simulink model "Hopper_GMEKF"  (R2026a)
settings: Solver=FixedStepAuto
settings Model: DataDictionary=NavigationDictionary.sldd  Creator=David  LastModifiedBy=David

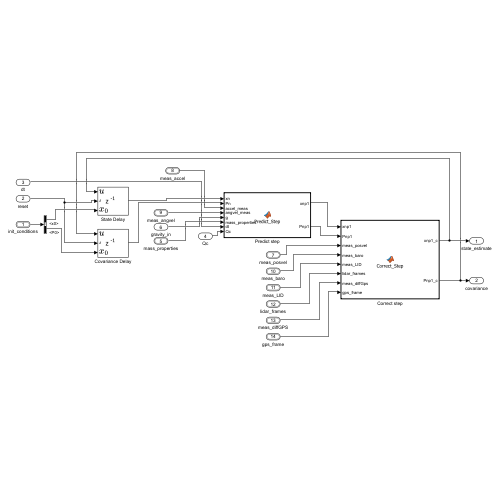
[thumbnail: Simulink's stored preview of the top-level diagram]
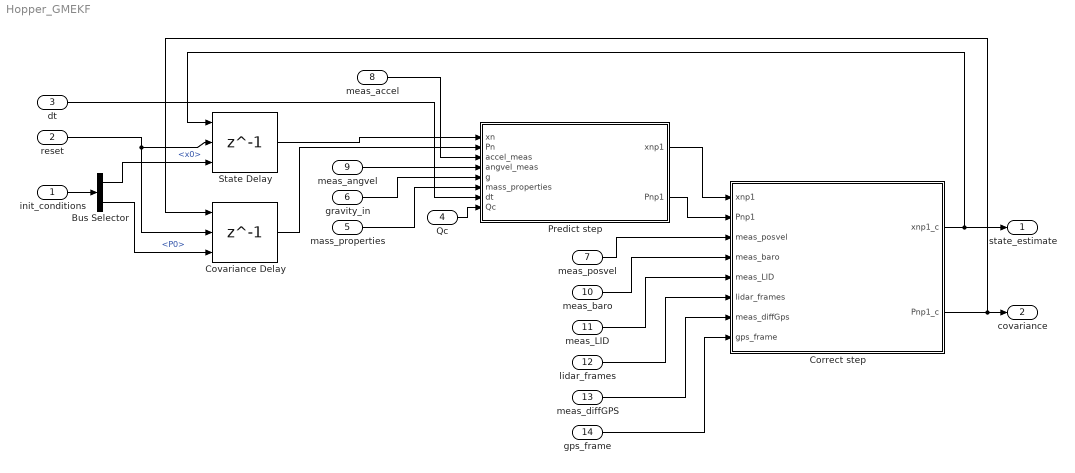
== system Hopper_GMEKF ==
  init_conditions : Inport  OutDataTypeStr=Bus: InitConditions
  reset : Inport  Port=2  OutDataTypeStr=ValueType: reset
  dt : Inport  Port=3  OutDataTypeStr=ValueType: timestep
  Qc : Inport  Port=4  OutDataTypeStr=ValueType: Qc
  mass_properties : Inport  Port=5  OutDataTypeStr=Bus: massProperties
  gravity_in : Inport  Port=6  OutDataTypeStr=ValueType: gravity
  meas_posvel : Inport  Port=7  OutDataTypeStr=Bus: gpsBus
  meas_accel : Inport  Port=8  OutDataTypeStr=Bus: accelBus
  meas_angvel : Inport  Port=9  OutDataTypeStr=Bus: angvelBus
  meas_baro : Inport  Port=10  OutDataTypeStr=Bus: baroBus
  meas_LID : Inport  Port=11  OutDataTypeStr=Bus: lidarBus
  lidar_frames : Inport  Port=12  OutDataTypeStr=Bus: lidarFrameBus
  meas_diffGPS : Inport  Port=13  OutDataTypeStr=Bus: diffGpsBus
  gps_frame : Inport  Port=14  OutDataTypeStr=Bus: gpsFrameBus
  Bus Selector : BusSelector  OutputSignals=x0,P0
  Correct step : MATLAB Function  TreatAsAtomicUnit=on  SystemSampleTime=1/500
  Covariance Delay : Delay  DelayLength=1  InitialConditionSource=Input port  ExternalReset=Rising
      settings: InputPortMap=u0,r5,p4
  Predict step : MATLAB Function  TreatAsAtomicUnit=on  SystemSampleTime=1/500
  State Delay : Delay  DelayLength=1  InitialConditionSource=Input port  ExternalReset=Rising
      settings: InputPortMap=u0,r5,p4
  state_estimate : Outport
  covariance : Outport  Port=2
  wires:
  init_conditions/1 -> Bus Selector/1
  Bus Selector/1 -> State Delay/3  "<x0>"
  Bus Selector/2 -> Covariance Delay/3  "<P0>"
  reset/1 -> Covariance Delay/2, State Delay/2
  State Delay/1 -> Predict step/1(xn)
  meas_accel/1 -> Predict step/3(accel_meas)
  dt/1 -> Predict step/7(dt)
  Covariance Delay/1 -> Predict step/2(Pn)
  gravity_in/1 -> Predict step/5(g)
  mass_properties/1 -> Predict step/6(mass_properties)
  Qc/1 -> Predict step/8(Qc)
  Predict step/1(xnp1) -> Correct step/1(xnp1)
  Predict step/2(Pnp1) -> Correct step/2(Pnp1)
  meas_posvel/1 -> Correct step/3(meas_posvel)
  meas_baro/1 -> Correct step/4(meas_baro)
  meas_LID/1 -> Correct step/5(meas_LID)
  lidar_frames/1 -> Correct step/6(lidar_frames)
  meas_diffGPS/1 -> Correct step/7(meas_diffGps)
  Correct step/2(Pnp1_c) -> Covariance Delay/1, covariance/1
  Correct step/1(xnp1_c) -> State Delay/1, state_estimate/1
  gps_frame/1 -> Correct step/8(gps_frame)
  meas_angvel/1 -> Predict step/4(angvel_meas)

== matlab function Hopper_GMEKF/Correct step ==
  data: xnp1 input size=[20 1]; xnp1_c output size=[20 1]; Pnp1 input size=[19 19]; meas_posvel input Bus: gpsBus; Pnp1_c output size=[19 19]; meas_baro input Bus: baroBus; meas_LID input Bus: lidarBus; lidar_frames input Bus: lidarFrameBus; meas_diffGps input Bus: diffGpsBus; gps_frame input Bus: gpsFrameBus
function [xnp1_c, Pnp1_c] = Correct_Step(xnp1, Pnp1, meas_posvel, meas_baro, meas_LID, lidar_frames, meas_diffGps, gps_frame)
[xnp1_c, Pnp1_c] = gmekf_correct_hopper(xnp1, Pnp1, meas_posvel, ...
    meas_baro, meas_LID, lidar_frames, meas_diffGps, gps_frame);
end

== matlab function Hopper_GMEKF/Predict step ==
  data: xn input size=[20 1]; Pn input size=[19 19]; xnp1 output size=[20 1]; accel_meas input Bus: accelBus; angvel_meas input Bus: angvelBus; g input size=1; mass_properties input Bus: massProperties; dt input size=1; Pnp1 output size=[19 19]; Qc input size=[13 13]
function [xnp1, Pnp1] = Predict_Step(xn, Pn, accel_meas, angvel_meas, g, mass_properties, dt, Qc)
% Unpack the structs
J = mass_properties.J;
accel = accel_meas.accel;
angvel = angvel_meas.angvel;
validity = accel_meas.validity;
[xnp1, Pnp1] = gmekf_predict(xn, Pn, accel, angvel, validity, J, g, dt, Qc);
end
